simulink model "new_fixed"  (R2024b)
settings: Solver=ode23t  StartTime=0.0  StopTime=2  MaxStep=1e-4  RelTol=1e-3  EnableMultiTasking=on
libraries: ee_lib x11, nesl_utility x7, fl_lib x3, simulink x2
CloseFcn:
  | clear simlog_IMStarting
  | clear logsout_IMStarting
Description:
  | Three-Phase Asynchronous Machine Starting
settings Model: Creator=The MathWorks, Inc.  LastModifiedBy=aminbgr
settings SolverCC: AlgebraicLoopSolver=TrustRegion  MaxZcPerStep=1
settings DataIOCC: LimitDataPoints=on  MaxDataPoints=90000  SaveFormat=Array  SaveOutput=off  SignalLogging=off  ReturnWorkspaceOutputs=off  SignalLoggingName=logsout_IMStarting
settings OptimizationCC: ReuseModelBlockBuffer=off  LifeSpan=inf
settings DebuggingCC: UnconnectedInputMsg=warning  UnconnectedOutputMsg=warning  UnconnectedLineMsg=warning  SFUnexpectedBacktrackingDiag=warning  SFNoUnconditionalDefaultTransitionDiag=warning  SFExecutionAtInitializationDiag=none  ArithmeticOperatorsInVariantConditions=warning
settings HardwareCC: ProdBitPerPointer=32  ProdBitPerSizeT=32  ProdBitPerPtrDiffT=32  ProdLargestAtomicFloat=None  ProdIntDivRoundTo=Undefined  ProdEndianess=Unspecified  ProdWordSize=32  ProdHWDeviceType=32-bit Generic
settings ModelReferenceCC: EnableRefExpFcnMdlSchedulingChecks=on  PropagateSignalLabelsOutOfModel=off
settings SFSimCC: SimUseLocalCustomCode=off  CustomCodeUndefinedFunction=UseInterfaceOnly
settings RTWCC: RTWUseLocalCustomCode=off  GPUComputeCapability=3.5  DLArmComputeVersion=19.05
settings CodeAppCC: StateflowObjectComments=on
settings GRTTargetCC: TargetLangStandard=C89/C90 (ANSI)
settings ConfigComp: CovMetricSettings=dw  CovSaveCumulativeToWorkspaceVar=on  CovSaveSingleToWorkspaceVar=on  CovExternalEMLEnable=off  CovSFcnEnable=off
settings SimscapeCC: SimscapeLogType=all  SimscapeLogSimulationStatistics=on  SimscapeLogName=simlog_IMStarting  SimscapeLogDataHistory=90000

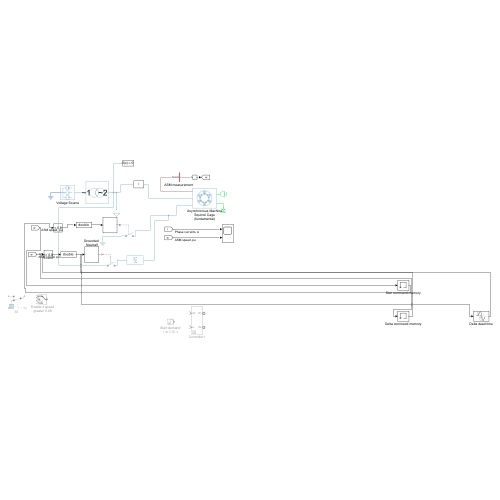
[thumbnail: Simulink's stored preview of the top-level diagram]
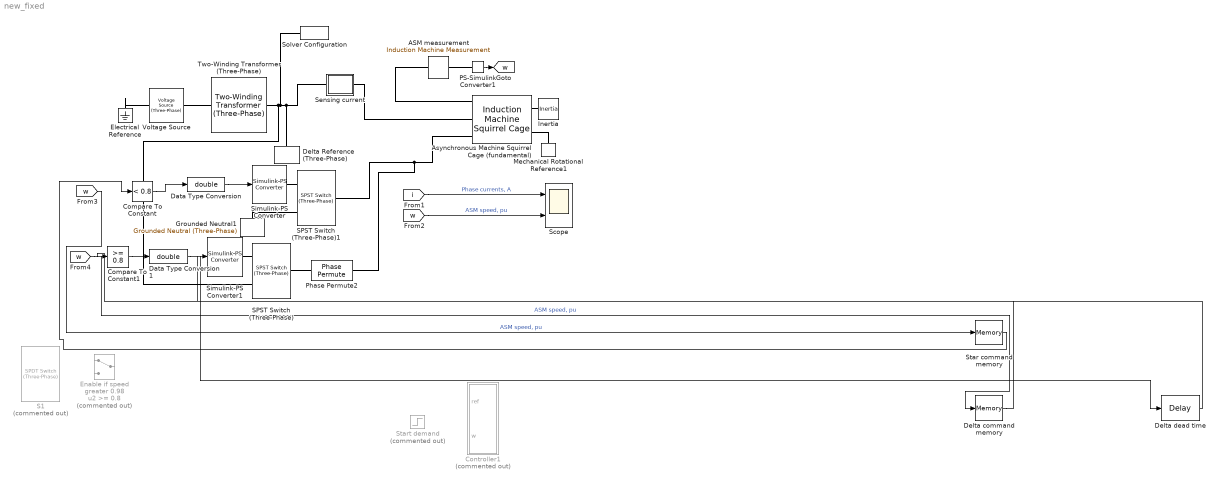
== system new_fixed ==
  ASM measurement : ee_lib/Electromechanical/Asynchronous/Induction Machine Measurement  output_idx=2
      settings: InternalSimscapePortConfiguration="{\"Bottom\":[],\"Left\":[{\"id\":\"pu_input\",\"label\":\"pu\",\"type\":\"input\"}],\"Right\":[{\"id\":\"pu_output\",\"label\":\"o\",\"type\":\"output\"}],\"Top\":[]}"
  Asynchronous Machine Squirrel Cage (fundamental) : ee_lib/Electromechanical/Asynchronous/Induction Machine Squirrel Cage  port_option=ee.enum.threePhasePort.composite  SRated=105308.6891 V*A  VRated=400 V  FRated=50 Hz  nPolePairs=1  param_unit=ee.enum.unit.si  squirrel_cage=ee.enum.squirrelcage.Double  zero_sequence=ee.enum.park.zerosequence.exclude  initialization_option=ee.enum.asm.initialization.fluxvariables  Rs=0.05751 Ohm  Xls=0.0606013222877 Ohm  pu_Rs=0.0258  pu_Lls=0.0413  Rrd=0.14 Ohm  Xlrd=0.41 Ohm  pu_Rrd=0.0145  pu_Llrd=0.0424  Rrd1=0.01311 Ohm  Xlrd1=0.166347331008 Ohm  Rrd2=0.305 Ohm  Xlrd2=0.0606013222877 Ohm  pu_Rrd1=0.0290  pu_Llrd1=0.0848  pu_Rrd2=0.0290  pu_Llrd2=0.0848  Xm=4.38252175176 Ohm  pu_Lm=1.7562  X0=0.4 Ohm  pu_L0=0.0413  saturation_option=ee.enum.saturation.include  saturation_i=[0, 4, 9, 18, 25, 34, 50, 68, 95, 120] A  saturation_v=[0, 88, 154, 198, 220, 242, 264, 286, 308, 327] V  pu_saturation_i=[0, .176, .396, .792, 1.1, 1.496, 2.2, 2.992, 4.18, 5.28]  pu_saturation_v=[0, .4, .7, .9, 1, 1.1, 1.2, 1.3, 1.4, 1.4864]  connection_option=ee.enum.Connection.delta1  angular_position_specify=off  angular_position_priority=None  angular_position=0 deg  angular_position_nominal_specify=off  angular_position_nominal_value=1  angular_position_nominal_unit=deg  pu_psids_specify=off  pu_psids_priority=None  pu_psids=0  pu_psids_nominal_specify=off  pu_psids_nominal_value=1  pu_psids_nominal_unit=1  pu_psiqs_specify=off  pu_psiqs_priority=None  pu_psiqs=0  pu_psiqs_nominal_specify=off  pu_psiqs_nominal_value=1  pu_psiqs_nominal_unit=1  pu_psi0s_specify=off  pu_psi0s_priority=None  pu_psi0s=0  pu_psi0s_nominal_specify=off  pu_psi0s_nominal_value=1  pu_psi0s_nominal_unit=1  pu_psidr_specify=off  pu_psidr_priority=None  pu_psidr=0  pu_psidr_nominal_specify=off  pu_psidr_nominal_value=1  pu_psidr_nominal_unit=1  pu_psiqr_specify=off  pu_psiqr_priority=None  pu_psiqr=0  pu_psiqr_nominal_specify=off  pu_psiqr_nominal_value=1  pu_psiqr_nominal_unit=1  pu_psidr1_specify=off  pu_psidr1_priority=None  pu_psidr1=0  pu_psidr1_nominal_specify=off  pu_psidr1_nominal_value=1  pu_psidr1_nominal_unit=1  pu_psiqr1_specify=off  pu_psiqr1_priority=None  pu_psiqr1=0  pu_psiqr1_nominal_specify=off  pu_psiqr1_nominal_value=1  pu_psiqr1_nominal_unit=1  pu_psidr2_specify=off  pu_psidr2_priority=None  pu_psidr2=0  pu_psidr2_nominal_specify=off  pu_psidr2_nominal_value=1  pu_psidr2_nominal_unit=1  pu_psiqr2_specify=off  pu_psiqr2_priority=None  pu_psiqr2=0  pu_psiqr2_nominal_specify=off  pu_psiqr2_nominal_value=1  pu_psiqr2_nominal_unit=1  psids_specify=off  psids_priority=None  psids=0 Wb  psids_nominal_specify=off  psids_nominal_value=1  psids_nominal_unit=Wb  psiqs_specify=off  psiqs_priority=None  psiqs=0 Wb  psiqs_nominal_specify=off  psiqs_nominal_value=1  psiqs_nominal_unit=Wb  psi0s_specify=off  psi0s_priority=None  psi0s=0 Wb  psi0s_nominal_specify=off  psi0s_nominal_value=1  psi0s_nominal_unit=Wb  psidr_specify=off  psidr_priority=None  psidr=0 Wb  psidr_nominal_specify=off  psidr_nominal_value=1  psidr_nominal_unit=Wb  psiqr_specify=off  psiqr_priority=None  psiqr=0 Wb  psiqr_nominal_specify=off  psiqr_nominal_value=1  psiqr_nominal_unit=Wb  psidr1_specify=off  psidr1_priority=None  psidr1=0 Wb  psidr1_nominal_specify=off  psidr1_nominal_value=1  psidr1_nominal_unit=Wb  psiqr1_specify=off  psiqr1_priority=None  psiqr1=0 Wb  psiqr1_nominal_specify=off  psiqr1_nominal_value=1  psiqr1_nominal_unit=Wb  psidr2_specify=off  psidr2_priority=None  psidr2=0 Wb  psidr2_nominal_specify=off  psidr2_nominal_value=1  psidr2_nominal_unit=Wb  psiqr2_specify=off  psiqr2_priority=None  psiqr2=0 Wb  psiqr2_nominal_specify=off  psiqr2_nominal_value=1  psiqr2_nominal_unit=Wb  slip_specify=off  slip_priority=None  slip=0  slip_nominal_specify=off  slip_nominal_value=1  slip_nominal_unit=1  real_power_generated_specify=off  real_power_generated_priority=None  real_power_generated=0 W  real_power_generated_nominal_specify=off  real_power_generated_nominal_value=1  real_power_generated_nominal_unit=W  mechanical_power_consumed_specify=off  mechanical_power_consumed_priority=None  mechanical_power_consumed=0 W  mechanical_power_consumed_nominal_specify=off  mechanical_power_consumed_nominal_value=1  mechanical_power_consumed_nominal_unit=W  Tmeas=298.15 K  alpha=3.93e-3 1/K  alpha_cage=4.4e-3 1/K  stator_thermal_mass=100 J/K  rotor_thermal_mass=200 J/K  temperatureA_specify=off  temperatureA_priority=High  temperatureA=25 degC  temperatureA_nominal_specify=off  temperatureA_nominal_value=1  temperatureA_nominal_unit=degC  temperatureB_specify=off  temperatureB_priority=High  temperatureB=25 degC  temperatureB_nominal_specify=off  temperatureB_nominal_value=1  temperatureB_nominal_unit=degC  temperatureC_specify=off  temperatureC_priority=High  temperatureC=25 degC  temperatureC_nominal_specify=off  temperatureC_nominal_value=1  temperatureC_nominal_unit=degC  temperatureR_specify=off  temperatureR_priority=High  temperatureR=25 degC  temperatureR_nominal_specify=off  temperatureR_nominal_value=1  temperatureR_nominal_unit=degC
      settings: InternalSimscapePortConfiguration="{\"Bottom\":[],\"Left\":[{\"id\":\"R\",\"label\":\"R\",\"type\":\"foundation.mechanical.rotational.rotational\"},{\"id\":\"C\",\"label\":\"C\",\"type\":\"foundation.mechanical.rotational.rotational\"}],\"Right\":[{\"id\":\"pu_output\",\"label\":\"pu\",\"type\":\"output\"},{\"id\":\"N1\",\"label\":\"~1\",\"type\":\"foundation.electrical.three_phase\"},{\"id\":\"N2\",\"label\":\"~2\",\"type\":\"foundation.electrical.three_phase\"}],\"Top\":[]}"
  Compare To Constant : simulink/Logic and Bit Operations/Compare To Constant  relop=<  const=0.8  OutDataTypeStr=boolean
  Compare To Constant1 : simulink/Logic and Bit Operations/Compare To Constant  relop=>=  const=0.8  OutDataTypeStr=boolean
  Controller1 : Subsystem  Commented=on
  Data Type Conversion : DataTypeConversion  OutDataTypeStr=double  SaturateOnIntegerOverflow=off  RndMeth=Floor
  Data Type Conversion1 : DataTypeConversion  OutDataTypeStr=double  SaturateOnIntegerOverflow=off  RndMeth=Floor
  Delta Reference (Three-Phase) : ee_lib/Connectors & References/Delta Reference (Three-Phase)
      settings: InternalSimscapePortConfiguration="{\"Bottom\":[],\"Left\":[{\"id\":\"N\",\"label\":\"~\",\"type\":\"foundation.electrical.three_phase\"}],\"Right\":[],\"Top\":[]}"
  Delta command memory : Memory
  Delta dead time : TransportDelay  DelayTime=0.03
  Electrical Reference : fl_lib/Electrical/Electrical Elements/Electrical Reference
  Enable if speed greater 0.98 : Switch  Commented=on  Threshold=0.8  SaturateOnIntegerOverflow=off  InputSameDT=off
  Grounded Neutral1 : ee_lib/Connectors & References/Grounded Neutral (Three-Phase)
  Inertia : fl_lib/Mechanical/Rotational Elements/Inertia  inertia=0.94 kg*m^2  num_ports=foundation.enum.numPorts2.one  w_specify=off  w_priority=High  w=0 rad/s  w_nominal_specify=off  w_nominal_value=1  w_nominal_unit=rad/s  t_specify=off  t_priority=High  t=0 N*m  t_nominal_specify=off  t_nominal_value=1  t_nominal_unit=N*m
  Mechanical Rotational Reference1 : fl_lib/Mechanical/Rotational Elements/Mechanical Rotational Reference
  PS-Simulink Converter1 : nesl_utility/PS-Simulink Converter  PhysicalDomain=network_engine_domain  SubClassName=ps_output  LeftPortType=input  RightPortType=output  PseudoPeriodic=off  Frequencies=[]  VectorFormat=1-D array  Unit=1  AffineConversion=off
  Phase Permute2 : ee_lib/Connectors & References/Phase Permute
      settings: InternalSimscapePortConfiguration="{\"Bottom\":[],\"Left\":[{\"id\":\"N123\",\"label\":\"~123\",\"type\":\"foundation.electrical.three_phase\"}],\"Right\":[{\"id\":\"N231\",\"label\":\"~231\",\"type\":\"foundation.electrical.three_phase\"}],\"Top\":[]}"
  S1 : ee_lib/Switches & Breakers/SPDT Switch (Three-Phase)  Commented=on  R_closed=0.001 Ohm  G_open=1e-6 1/Ohm  threshold=0.5 V  i_vT_specify=off  i_vT_priority=None  i_vT=0 A  i_vT_nominal_specify=off  i_vT_nominal_value=1  i_vT_nominal_unit=A  I12_specify=off  I12_priority=None  I12=[ 0 0 0 ] A  I12_nominal_specify=off  I12_nominal_value=1  I12_nominal_unit=A  V12_specify=off  V12_priority=None  V12=[ 0 0 0 ] V  V12_nominal_specify=off  V12_nominal_value=1  V12_nominal_unit=V  I13_specify=off  I13_priority=None  I13=[ 0 0 0 ] A  I13_nominal_specify=off  I13_nominal_value=1  I13_nominal_unit=A  V13_specify=off  V13_priority=None  V13=[ 0 0 0 ] V  V13_nominal_specify=off  V13_nominal_value=1  V13_nominal_unit=V  i_a_12_specify=off  i_a_12_priority=None  i_a_12=0 A  i_a_12_nominal_specify=off  i_a_12_nominal_value=1  i_a_12_nominal_unit=A  v_a_12_specify=off  v_a_12_priority=None  v_a_12=0 V  v_a_12_nominal_specify=off  v_a_12_nominal_value=1  v_a_12_nominal_unit=V  i_a_13_specify=off  i_a_13_priority=None  i_a_13=0 A  i_a_13_nominal_specify=off  i_a_13_nominal_value=1  i_a_13_nominal_unit=A  v_a_13_specify=off  v_a_13_priority=None  v_a_13=0 V  v_a_13_nominal_specify=off  v_a_13_nominal_value=1  v_a_13_nominal_unit=V  i_b_12_specify=off  i_b_12_priority=None  i_b_12=0 A  i_b_12_nominal_specify=off  i_b_12_nominal_value=1  i_b_12_nominal_unit=A  v_b_12_specify=off  v_b_12_priority=None  v_b_12=0 V  v_b_12_nominal_specify=off  v_b_12_nominal_value=1  v_b_12_nominal_unit=V  i_b_13_specify=off  i_b_13_priority=None  i_b_13=0 A  i_b_13_nominal_specify=off  i_b_13_nominal_value=1  i_b_13_nominal_unit=A  v_b_13_specify=off  v_b_13_priority=None  v_b_13=0 V  v_b_13_nominal_specify=off  v_b_13_nominal_value=1  v_b_13_nominal_unit=V  i_c_12_specify=off  i_c_12_priority=None  i_c_12=0 A  i_c_12_nominal_specify=off  i_c_12_nominal_value=1  i_c_12_nominal_unit=A  v_c_12_specify=off  v_c_12_priority=None  v_c_12=0 V  v_c_12_nominal_specify=off  v_c_12_nominal_value=1  v_c_12_nominal_unit=V  i_c_13_specify=off  i_c_13_priority=None  i_c_13=0 A  i_c_13_nominal_specify=off  i_c_13_nominal_value=1  i_c_13_nominal_unit=A  v_c_13_specify=off  v_c_13_priority=None  v_c_13=0 V  v_c_13_nominal_specify=off  v_c_13_nominal_value=1  v_c_13_nominal_unit=V
      settings: InternalSimscapePortConfiguration="{\"Bottom\":[],\"Left\":[{\"id\":\"vT\",\"label\":\"vT\",\"type\":\"input\"},{\"id\":\"N1\",\"label\":\"~1\",\"type\":\"foundation.electrical.three_phase\"}],\"Right\":[{\"id\":\"N2\",\"label\":\"~2\",\"type\":\"foundation.electrical.three_phase\"},{\"id\":\"N3\",\"label\":\"~3\",\"type\":\"foundation.electrical.three_phase\"}],\"Top\":[]}"
  SPST Switch (Three-Phase) : ee_lib/Switches & Breakers/SPST Switch (Three-Phase)  R_closed=0.001 Ohm  G_open=1e-6 1/Ohm  threshold=0.5 V  i_vT_specify=off  i_vT_priority=None  i_vT=0 A  i_vT_nominal_specify=off  i_vT_nominal_value=1  i_vT_nominal_unit=A  I_specify=off  I_priority=None  I=[0, 0, 0] A  I_nominal_specify=off  I_nominal_value=1  I_nominal_unit=A  V_specify=off  V_priority=None  V=[0, 0, 0] V  V_nominal_specify=off  V_nominal_value=1  V_nominal_unit=V  i_a_specify=off  i_a_priority=None  i_a=0 A  i_a_nominal_specify=off  i_a_nominal_value=1  i_a_nominal_unit=A  v_a_specify=off  v_a_priority=None  v_a=0 V  v_a_nominal_specify=off  v_a_nominal_value=1  v_a_nominal_unit=V  i_b_specify=off  i_b_priority=None  i_b=0 A  i_b_nominal_specify=off  i_b_nominal_value=1  i_b_nominal_unit=A  v_b_specify=off  v_b_priority=None  v_b=0 V  v_b_nominal_specify=off  v_b_nominal_value=1  v_b_nominal_unit=V  i_c_specify=off  i_c_priority=None  i_c=0 A  i_c_nominal_specify=off  i_c_nominal_value=1  i_c_nominal_unit=A  v_c_specify=off  v_c_priority=None  v_c=0 V  v_c_nominal_specify=off  v_c_nominal_value=1  v_c_nominal_unit=V
      settings: InternalSimscapePortConfiguration="{\"Bottom\":[],\"Left\":[{\"id\":\"vT\",\"label\":\"vT\",\"type\":\"input\"},{\"id\":\"N1\",\"label\":\"~1\",\"type\":\"foundation.electrical.three_phase\"}],\"Right\":[{\"id\":\"N2\",\"label\":\"~2\",\"type\":\"foundation.electrical.three_phase\"}],\"Top\":[]}"
  SPST Switch (Three-Phase)1 : ee_lib/Switches & Breakers/SPST Switch (Three-Phase)  R_closed=0.001 Ohm  G_open=1e-6 1/Ohm  threshold=0.5 V  i_vT_specify=off  i_vT_priority=None  i_vT=0 A  i_vT_nominal_specify=off  i_vT_nominal_value=1  i_vT_nominal_unit=A  I_specify=off  I_priority=None  I=[0, 0, 0] A  I_nominal_specify=off  I_nominal_value=1  I_nominal_unit=A  V_specify=off  V_priority=None  V=[0, 0, 0] V  V_nominal_specify=off  V_nominal_value=1  V_nominal_unit=V  i_a_specify=off  i_a_priority=None  i_a=0 A  i_a_nominal_specify=off  i_a_nominal_value=1  i_a_nominal_unit=A  v_a_specify=off  v_a_priority=None  v_a=0 V  v_a_nominal_specify=off  v_a_nominal_value=1  v_a_nominal_unit=V  i_b_specify=off  i_b_priority=None  i_b=0 A  i_b_nominal_specify=off  i_b_nominal_value=1  i_b_nominal_unit=A  v_b_specify=off  v_b_priority=None  v_b=0 V  v_b_nominal_specify=off  v_b_nominal_value=1  v_b_nominal_unit=V  i_c_specify=off  i_c_priority=None  i_c=0 A  i_c_nominal_specify=off  i_c_nominal_value=1  i_c_nominal_unit=A  v_c_specify=off  v_c_priority=None  v_c=0 V  v_c_nominal_specify=off  v_c_nominal_value=1  v_c_nominal_unit=V
      settings: InternalSimscapePortConfiguration="{\"Bottom\":[],\"Left\":[{\"id\":\"vT\",\"label\":\"vT\",\"type\":\"input\"},{\"id\":\"N1\",\"label\":\"~1\",\"type\":\"foundation.electrical.three_phase\"}],\"Right\":[{\"id\":\"N2\",\"label\":\"~2\",\"type\":\"foundation.electrical.three_phase\"}],\"Top\":[]}"
  Scope : Scope  NumInputPorts=2
  Sensing current : Subsystem
      mask Display: disp('i')
  Simulink-PS Converter : nesl_utility/Simulink-PS Converter  PhysicalDomain=network_engine_domain  SubClassName=ps_input  LeftPortType=input  RightPortType=output  PseudoPeriodic=off  Frequencies=[]  NoiseDistribution=none  NoiseParameters=[]  Unit=1  AffineConversion=off  FilteringAndDerivatives=provide  SimscapeFilterOrder=1  InputFilterTimeConstant=0.001  UdotUserProvided=0
  Simulink-PS Converter1 : nesl_utility/Simulink-PS Converter  PhysicalDomain=network_engine_domain  SubClassName=ps_input  LeftPortType=input  RightPortType=output  PseudoPeriodic=off  Frequencies=[]  NoiseDistribution=none  NoiseParameters=[]  Unit=1  AffineConversion=off  FilteringAndDerivatives=provide  SimscapeFilterOrder=1  InputFilterTimeConstant=0.001  UdotUserProvided=0
  Solver Configuration : nesl_utility/Solver Configuration  PhysicalDomain=network_engine_domain  SubClassName=solver  LeftPortType=input  RightPortType=generic  Tones=[]  Harmonics=[]  SimulateNoise=off  Profile=off  UseLocalSampling=off  EnableSwitchedLinearOptims=on  FrequencyDomain=off  UseCCode=off  RelTol=0.001  AbsTol=1e-06  MinStep=1e-09  ToWorkspace=off  RevertToSquareIcSolve=off  NumHomotopyIterations=100  PhasorMode=off  PhasorModeNumHarmonics=1  ConsistencySolver=NEWTON_FTOL  IndexReductionMethod=DerivativeReplacement  DoDC=off  ResidualTolerance=1e-9  ConsistencyTolSource=GLOBAL  ConsistencyAbsTol=0.001  ConsistencyRelTol=0.001  ConsistencyTolFactor=0.001  UseLocalSolver=on  LocalSolverChoice=NE_BACKWARD_EULER_ADVANCER  ResolveIndetEquations=on  FunctionEvalNumThread=1  LocalSolverSampleTime=1e-4  DoFixedCost=off  MaxNonlinIter=3  MaxModeIter=2  ComputeImpulses=off  ImpulseIterations=2  LinearAlgebra=auto  LinearAlgebraNumThread=0  EquationFormulation=NE_TIME_EF  DelaysMemoryBudget=1024  AutomaticFiltering=on  FilteringTimeConstant=0.001  PartitionStorageMethod=AS_NEEDED  PartitionMemoryBudget=1024  PartitionMethod=FAST  MultibodyUseLocalSolver=off  MultibodyLocalSolverChoice=ODE1  MultibodyLocalSolverSampleTime=0.001
  Star command memory : Memory
  Start demand : Step  Commented=on  Time=0.05  SampleTime=0
      settings: AttributesFormatString=%<After> at %<Time> s
  Two-Winding Transformer (Three-Phase) : ee_lib/Passive/Transformers/Two-Winding Transformer (Three-Phase)  SRated=125e+3 A*V  FRated=50 Hz  Winding1Connection=ee.enum.windingconnection.Yg  VRated1=20e+3 V  Winding2Connection=ee.enum.windingconnection.delta1  VRated2=400 V  CoreType=ee.enum.coretype.threelimb  pu_Rw1=0.005  pu_Rw2=0.005  leakage_reactance_option=ee.enum.transformer_leakage.include  pu_Xl1=0.05  pu_Xl2=0.05  magnetizing_resistance_option=ee.enum.transformer_magnetizingResistance.include  pu_Rm=500  magnetizing_reactance_option=ee.enum.transformer_magnetizingReactance.exclude  saturation_option=ee.enum.transformer_saturation.exclude  pu_Xm=500  current_data=[0, .002, 1, 2]  magnetic_flux_data=[0, 1.2, 1.5, 1.51]  pu_X0=0.5  i1_specify=off  i1_priority=None  i1=[0, 0, 0] A  i1_nominal_specify=off  i1_nominal_value=1  i1_nominal_unit=A  i2_specify=off  i2_priority=None  i2=[0, 0, 0] A  i2_nominal_specify=off  i2_nominal_value=1  i2_nominal_unit=A  phi_specify=off  phi_priority=None  phi=[0, 0, 0]  phi_nominal_specify=off  phi_nominal_value=1  phi_nominal_unit=1  power_dissipated_specify=off  power_dissipated_priority=None  power_dissipated=0 W  power_dissipated_nominal_specify=off  power_dissipated_nominal_value=1  power_dissipated_nominal_unit=W
      settings: InternalSimscapePortConfiguration="{\"Bottom\":[],\"Left\":[{\"id\":\"N1\",\"label\":\"~1\",\"type\":\"foundation.electrical.three_phase\"}],\"Right\":[{\"id\":\"N2\",\"label\":\"~2\",\"type\":\"foundation.electrical.three_phase\"}],\"Top\":[]}"
  Voltage Source : ee_lib/Sources/Voltage Source (Three-Phase)  vline_rms=20e3 V  shift=0 deg  freq=50 Hz  impedance_option=2  SShortCircuit=20e6 V*A  XR=10  R=0.5 Ohm  L=3.97e-4 H  harmonic_option=0  harmonic_orders=[5, 7, 11, 13]  harmonic_ratios=[0.1, 0.1, 0.1, 0.1]  G_parasitic=0 1/Ohm  I_specify=off  I_priority=None  I=[ 0 0 0 ] A  I_nominal_specify=off  I_nominal_value=1  I_nominal_unit=A
  tag scope: w=global
  wires:
  PS-Simulink Converter1/1 -> [w]
  [i] -> Scope/1  "Phase currents, A"
  [w] -> Scope/2  "ASM speed, pu"
  Compare To Constant/1 -> Data Type Conversion/1
  Data Type Conversion/1 -> Simulink-PS Converter/1
  Compare To Constant1/1 -> Data Type Conversion1/1
  [w] -> Star command memory/1  "ASM speed, pu"
  Star command memory/1 -> Compare To Constant/1
  [w] -> Delta command memory/1  "ASM speed, pu"
  Delta command memory/1 -> Compare To Constant1/1
  Data Type Conversion1/1 -> Delta dead time/1
  Delta dead time/1 -> Simulink-PS Converter1/1
  connections:
  Asynchronous Machine Squirrel Cage (fundamental)/LConn1 -- Inertia/LConn1
  Mechanical Rotational Reference1/LConn1 -- Asynchronous Machine Squirrel Cage (fundamental)/LConn2
  Electrical Reference/LConn1 -- Voltage Source/LConn1
  Sensing current/RConn1 -- Asynchronous Machine Squirrel Cage (fundamental)/RConn2
  Asynchronous Machine Squirrel Cage (fundamental)/RConn1 -- ASM measurement/LConn1
  ASM measurement/RConn1 -- PS-Simulink Converter1/LConn1
  Two-Winding Transformer (Three-Phase)/RConn1 -- SPST Switch (Three-Phase)/LConn2 -- Solver Configuration/RConn1 -- Delta Reference (Three-Phase)/LConn1 -- Sensing current/LConn1
  Two-Winding Transformer (Three-Phase)/LConn1 -- Voltage Source/RConn1
  SPST Switch (Three-Phase)1/RConn1 -- Phase Permute2/RConn1 -- Asynchronous Machine Squirrel Cage (fundamental)/RConn3
  Grounded Neutral1/LConn1 -- SPST Switch (Three-Phase)1/LConn2
  Phase Permute2/LConn1 -- SPST Switch (Three-Phase)/RConn1
  Simulink-PS Converter/RConn1 -- SPST Switch (Three-Phase)1/LConn1
  Simulink-PS Converter1/RConn1 -- SPST Switch (Three-Phase)/LConn1

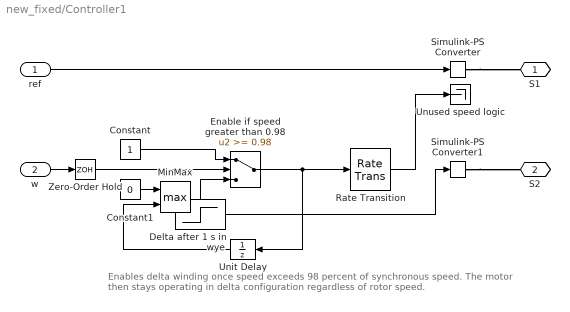
== system new_fixed/Controller1 ==
  note: Enables delta winding once speed exceeds 98 percent of synchronous
      | speed. The motor then stays operating in delta configuration regardless
      | of rotor speed.
  ref : Inport
  w : Inport  Port=2
  Constant : Constant
  Constant1 : Constant  Value=0
  Delta after 1 s in wye : Step  Time=1.05  SampleTime=0
  Enable if speed greater than 0.98 : Switch  Threshold=0.98  SaturateOnIntegerOverflow=off  InputSameDT=off
  MinMax : MinMax  Function=max  Inputs=2
  Rate Transition : RateTransition
  Simulink-PS Converter : nesl_utility/Simulink-PS Converter  PhysicalDomain=network_engine_domain  SubClassName=ps_input  LeftPortType=input  RightPortType=output  PseudoPeriodic=off  Frequencies=[]  NoiseDistribution=none  NoiseParameters=[]  Unit=1  AffineConversion=off  FilteringAndDerivatives=zero  SimscapeFilterOrder=1  InputFilterTimeConstant=0.001  UdotUserProvided=1
  Simulink-PS Converter1 : nesl_utility/Simulink-PS Converter  PhysicalDomain=network_engine_domain  SubClassName=ps_input  LeftPortType=input  RightPortType=output  PseudoPeriodic=off  Frequencies=[]  NoiseDistribution=none  NoiseParameters=[]  Unit=1  AffineConversion=off  FilteringAndDerivatives=zero  SimscapeFilterOrder=1  InputFilterTimeConstant=0.001  UdotUserProvided=1
  Unit Delay : UnitDelay  SampleTime=0.1  HasFrameUpgradeWarning=on
  Unused speed logic : Terminator
  Zero-Order Hold : ZeroOrderHold  SampleTime=0.1
  S1 : PMIOPort  Side=Right
  S2 : PMIOPort  Port=2  Side=Right
  wires:
  ref/1 -> Simulink-PS Converter/1
  Enable if speed greater than 0.98/1 -> Unit Delay/1, Rate Transition/1
  Constant/1 -> Enable if speed greater than 0.98/1
  w/1 -> Zero-Order Hold/1
  Zero-Order Hold/1 -> Enable if speed greater than 0.98/2
  MinMax/1 -> Enable if speed greater than 0.98/3
  Constant1/1 -> MinMax/1
  Unit Delay/1 -> MinMax/2
  Delta after 1 s in wye/1 -> Simulink-PS Converter1/1
  Rate Transition/1 -> Unused speed logic/1
  connections:
  Simulink-PS Converter/RConn1 -- S1/RConn1
  Simulink-PS Converter1/RConn1 -- S2/RConn1

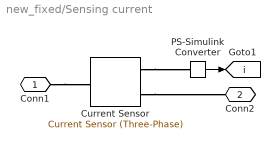
== system new_fixed/Sensing current ==
  Current Sensor : ee_lib/Sensors & Transducers/Current Sensor (Three-Phase)
  PS-Simulink Converter : nesl_utility/PS-Simulink Converter  PhysicalDomain=network_engine_domain  SubClassName=ps_output  LeftPortType=input  RightPortType=output  PseudoPeriodic=off  Frequencies=[]  VectorFormat=1-D array  Unit=1  AffineConversion=off
  Conn1 : PMIOPort  Side=Left
  Conn2 : PMIOPort  Port=2  Side=Right
  tag scope: i=global
  wires:
  PS-Simulink Converter/1 -> [i]
  connections:
  Current Sensor/RConn1 -- PS-Simulink Converter/LConn1
  Conn1/RConn1 -- Current Sensor/LConn1
  Current Sensor/RConn2 -- Conn2/RConn1
